simulink model "Stol_stabilizujacy_simulink"  (R2026b)
settings: Solver=VariableStepAuto  StopTime=t_end
values from neighbouring files (symbols this model uses):
  ball = m*g/(m + J_B/R^2)    (= 7.00714285714)    [Stol_stabilizujacy.m]
  Kd = 8/(9*b_deg*l_IMC)    (= 14.536475944)    [Stol_stabilizujacy.m]
  Kp = 1/(3*b_deg*l_IMC^2)    (= 10.902356958)    [Stol_stabilizujacy.m]
  N = 3/l_IMC    (= 6)    [Stol_stabilizujacy.m]
  r0 = 0.05    [Stol_stabilizujacy.m]
  r_zad = 0    [Stol_stabilizujacy.m]
  servoDamping = 1    [Stol_stabilizujacy.m]
  servoGain = 1    [Stol_stabilizujacy.m]
  servoTimeConstant = 0.05    [Stol_stabilizujacy.m]
  v0 = 0.02    [Stol_stabilizujacy.m]
settings Model: Creator=kacpe  LastModifiedBy=kacpe

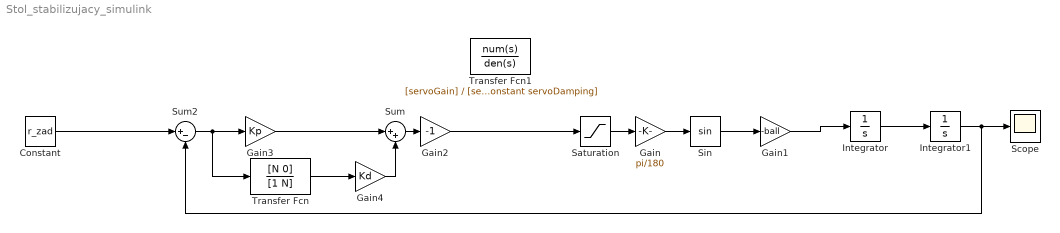
== system Stol_stabilizujacy_simulink ==
  Constant : Constant  Value=r_zad
  Gain : Gain  Gain=pi/180
  Gain1 : Gain  Gain=-ball
  Gain2 : Gain  Gain=-1
  Gain3 : Gain  Gain=Kp
  Gain4 : Gain  Gain=Kd
  Integrator : Integrator  InitialCondition=v0
  Integrator1 : Integrator  InitialCondition=r0
  Saturation : Saturate  UpperLimit=5  LowerLimit=-5
  Scope : Scope
      settings: ActiveDisplayYMinimum=-0.44729273930058822  ActiveDisplayYMaximum=0.49797331549060964
  Sin : Trigonometry
  Sum : Sum  Inputs=|++
  Sum2 : Sum  Inputs=|+-
  Transfer Fcn : TransferFcn  Numerator=[N 0]  Denominator=[1 N]
  Transfer Fcn1 : TransferFcn  Numerator=[servoGain]  Denominator=[servoTimeConstant servoDamping]
  wires:
  Gain/1 -> Sin/1
  Sin/1 -> Gain1/1
  Gain1/1 -> Integrator/1
  Integrator/1 -> Integrator1/1
  Integrator1/1 -> Sum2/2, Scope/1
  Constant/1 -> Sum2/1
  Sum2/1 -> Transfer Fcn/1, Gain3/1
  Transfer Fcn/1 -> Gain4/1
  Sum/1 -> Gain2/1
  Gain4/1 -> Sum/2
  Gain3/1 -> Sum/1
  Saturation/1 -> Gain/1
  Gain2/1 -> Saturation/1
